simulink library "tip_assist_lib_support"  (Simulink 9.0)
settings: Solver=VariableStepAuto  StartTime=0.0  StopTime=10.0  RelTol=1e-3
undefined symbols (not defined in the file): g, timestep, TipAssistAdvEcmError_t, TipAssistCpmTipOffMode_t, TipAssistLiveWeighStatus_t, TipAssistPayloadType_t, TipAssistSecPfwStatus_t, TipAssistUnsecPfwStatus_t, toa_appNumber, toa_expectedBucketAngNoise, toa_imu_lpf_cutoff_hz, toa_imuBasicOrient, toa_liftBoreDia, toa_liftRodDia, toa_liveLpfCutoffHz, toa_liveSpillRateLpfCutoffHz, toa_mcGroundCombBucketAng, toa_mcGroundCombLiftNormAng, toa_mcGroundLiftNormAng, toa_noSlidingAngle, toa_payload_target_ov_val, toa_payloadTargetMin, toa_pfwLpfCutoffHz, toa_pfwResetLpfCutoffHz, toa_pfwResetStatsBound, toa_pfwResetStatsConf, toa_pfwTiltNormRackThresh, toa_pfwTravelExtentLower, toa_pfwTravelExtentUpper, toa_ratedPayload, toa_reposeMarginAng, toa_sendCpmLiveLpfCutoffHz, toa_sendToCpmMinPrecision, toa_tiltBoreDia, toa_tiltNumCyl, toa_tiltRodDia, toa_toolBcAngle, toa_toolBcLength
libraries: lib_CATutils_Utilities_ApplyName_v2 x113, simulink x18, tip_assist_lib x14, lib_CATutils_Filters_1Pole_LowPass x6, simulink_extras x5, lib_CATutils_Override x3, lib_CATutils_Hysteresis_Latch x3, lib_CATutils_Timer_Countdown x3, tip_assist_lib_support x2
(part 2 of 4)

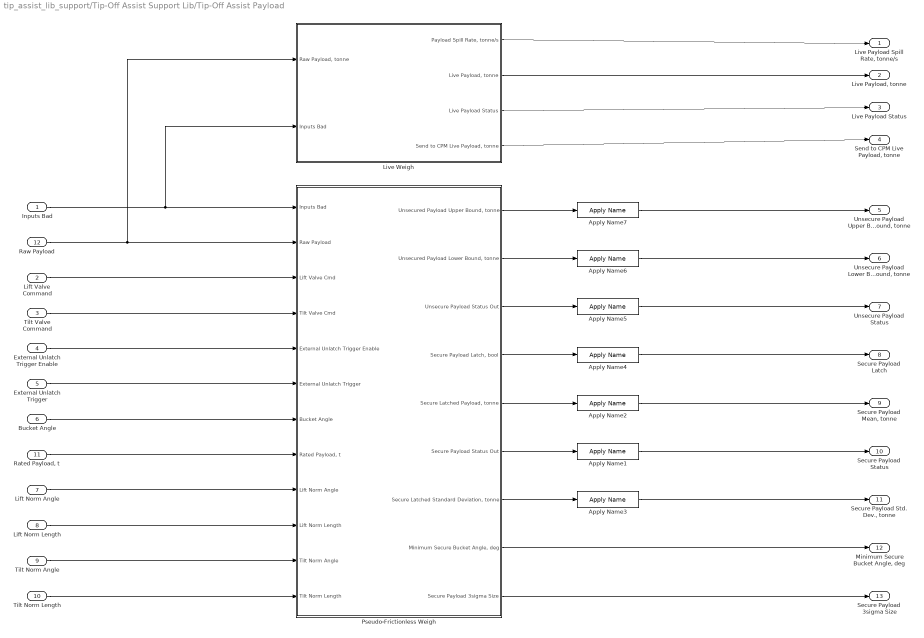
== system tip_assist_lib_support/Tip-Off Assist Support Lib/Tip-Off Assist Payload ==
  Inputs Bad : Inport
  Lift Valve Command : Inport  Port=2
  Tilt Valve Command : Inport  Port=3
  External Unlatch Trigger Enable : Inport  Port=4
  External Unlatch Trigger : Inport  Port=5
  Bucket Angle : Inport  Port=6
  Lift Norm Angle : Inport  Port=7
  Lift Norm Length : Inport  Port=8
  Tilt Norm Angle : Inport  Port=9
  Tilt Norm Length : Inport  Port=10
  "Rated Payload, t" : Inport  Port=11
  Raw Payload : Inport  Port=12
  Apply Name1 : lib_CATutils_Utilities_ApplyName_v2/Apply Name  sigLabel='toa_pfwSecStatus'  enTst=true
  Apply Name2 : lib_CATutils_Utilities_ApplyName_v2/Apply Name  sigLabel='toa_pfwSecPayload'  enTst=true
  Apply Name3 : lib_CATutils_Utilities_ApplyName_v2/Apply Name  sigLabel='toa_pfwSecStDev'  enTst=true
  Apply Name4 : lib_CATutils_Utilities_ApplyName_v2/Apply Name  sigLabel='toa_pfwSecLatch'  enTst=true
  Apply Name5 : lib_CATutils_Utilities_ApplyName_v2/Apply Name  sigLabel='toa_pfwUnsecStatus'  enTst=true
  Apply Name6 : lib_CATutils_Utilities_ApplyName_v2/Apply Name  sigLabel='toa_pfwUnsecBoundLower'  enTst=true
  Apply Name7 : lib_CATutils_Utilities_ApplyName_v2/Apply Name  sigLabel='toa_pfwUnsecBoundUpper'  enTst=true
  Live Weigh : Subsystem
  Pseudo-Frictionless Weigh : Subsystem
  "Live Payload Spill Rate, tonne/s" : Outport
  "Live Payload, tonne" : Outport  Port=2
  Live Payload Status : Outport  Port=3
  "Send to CPM Live Payload, tonne" : Outport  Port=4
  "Unsecure Payload Upper Bound, tonne" : Outport  Port=5
  "Unsecure Payload Lower Bound, tonne" : Outport  Port=6
  Unsecure Payload Status : Outport  Port=7
  Secure Payload Latch : Outport  Port=8
  "Secure Payload Mean, tonne" : Outport  Port=9
  Secure Payload Status : Outport  Port=10
  "Secure Payload Std. Dev., tonne" : Outport  Port=11
  "Minimum Secure Bucket Angle, deg" : Outport  Port=12
  Secure Payload 3sigma Size : Outport  Port=13
  wires:
  Lift Valve Command/1 -> Pseudo-Frictionless Weigh/3(Lift Valve Cmd)
  Tilt Valve Command/1 -> Pseudo-Frictionless Weigh/4(Tilt Valve Cmd)
  Pseudo-Frictionless Weigh/7("Secure Latched Standard Deviation, tonne") -> Apply Name3/1
  Pseudo-Frictionless Weigh/6(Secure Payload Status Out) -> Apply Name1/1
  Pseudo-Frictionless Weigh/4("Secure Payload Latch, bool") -> Apply Name4/1
  Pseudo-Frictionless Weigh/5("Secure Latched Payload, tonne") -> Apply Name2/1
  Raw Payload/1 -> Live Weigh/1("Raw Payload, tonne"), Pseudo-Frictionless Weigh/2(Raw Payload)
  Inputs Bad/1 -> Live Weigh/2(Inputs Bad), Pseudo-Frictionless Weigh/1(Inputs Bad)
  Live Weigh/1("Payload Spill Rate, tonne/s") -> "Live Payload Spill Rate, tonne/s"/1
  Live Weigh/2("Live Payload, tonne") -> "Live Payload, tonne"/1
  Live Weigh/3(Live Payload Status) -> Live Payload Status/1
  External Unlatch Trigger Enable/1 -> Pseudo-Frictionless Weigh/5(External Unlatch Trigger Enable)
  External Unlatch Trigger/1 -> Pseudo-Frictionless Weigh/6(External Unlatch Trigger)
  Bucket Angle/1 -> Pseudo-Frictionless Weigh/7(Bucket Angle)
  Pseudo-Frictionless Weigh/2("Unsecured Payload Lower Bound, tonne") -> Apply Name6/1
  Pseudo-Frictionless Weigh/1("Unsecured Payload Upper Bound, tonne") -> Apply Name7/1
  "Rated Payload, t"/1 -> Pseudo-Frictionless Weigh/8("Rated Payload, t")
  Lift Norm Angle/1 -> Pseudo-Frictionless Weigh/9("Lift Norm Angle ")
  Lift Norm Length/1 -> Pseudo-Frictionless Weigh/10(Lift Norm Length)
  Tilt Norm Angle/1 -> Pseudo-Frictionless Weigh/11(Tilt Norm Angle)
  Tilt Norm Length/1 -> Pseudo-Frictionless Weigh/12(Tilt Norm Length)
  Pseudo-Frictionless Weigh/3(Unsecure Payload Status Out) -> Apply Name5/1
  Apply Name4/1 -> Secure Payload Latch/1
  Apply Name2/1 -> "Secure Payload Mean, tonne"/1
  Apply Name1/1 -> Secure Payload Status/1
  Apply Name3/1 -> "Secure Payload Std. Dev., tonne"/1
  Apply Name5/1 -> Unsecure Payload Status/1
  Apply Name6/1 -> "Unsecure Payload Lower Bound, tonne"/1
  Apply Name7/1 -> "Unsecure Payload Upper Bound, tonne"/1
  Pseudo-Frictionless Weigh/8("Minimum Secure Bucket Angle, deg") -> "Minimum Secure Bucket Angle, deg"/1
  Pseudo-Frictionless Weigh/9(Secure Payload 3sigma Size) -> Secure Payload 3sigma Size/1
  Live Weigh/4("Send to CPM Live Payload, tonne") -> "Send to CPM Live Payload, tonne"/1

== system tip_assist_lib_support/Tip-Off Assist Support Lib/EEF IMU to NEEF gravity vector/imu lpf x1 ==
  in : Inport
  "cutoff freq, Hz" : Inport  Port=2
  Filter Factor Calc : Subsystem
  Single Pole Low Pass Filter : lib_CATutils_Filters_1Pole_LowPass/Single Pole Low Pass Filter  extFactor=on  extReset=off  incIntWordSize=off  mainInternalRes=off  filtFactor=.0001
  Single Pole Low Pass Filter1 : lib_CATutils_Filters_1Pole_LowPass/Single Pole Low Pass Filter  extFactor=on  extReset=off  incIntWordSize=off  mainInternalRes=off  filtFactor=.0001
  out : Outport
  wires:
  in/1 -> Single Pole Low Pass Filter/1
  Single Pole Low Pass Filter1/1 -> out/1
  Single Pole Low Pass Filter/1 -> Single Pole Low Pass Filter1/1
  "cutoff freq, Hz"/1 -> Filter Factor Calc/1(Cutoff (Hz))
  Filter Factor Calc/1(Filter Factor) -> Single Pole Low Pass Filter1/2, Single Pole Low Pass Filter/2

== system tip_assist_lib_support/Tip-Off Assist Support Lib/EEF IMU to NEEF gravity vector/normalize vector ==
  in : Inport
  Divide : Product  Inputs=*/  OutDataTypeStr=Inherit: Same as first input
  Math Function : Math  Operator=square  SaturateOnIntegerOverflow=on
  Math Function1 : Math  Operator=sqrt  SaturateOnIntegerOverflow=on
  Sum of Elements : Sum  Inputs=+
  out : Outport
  wires:
  Divide/1 -> out/1
  in/1 -> Math Function/1, Divide/1
  Math Function1/1 -> Divide/2
  Math Function/1 -> Sum of Elements/1
  Sum of Elements/1 -> Math Function1/1

== system tip_assist_lib_support/Tip-Off Assist Support Lib/Gravity Relevant Components/Magnitude ==
  vector : Inport
  Math Function : Math  Operator=square  SaturateOnIntegerOverflow=on
  Math Function1 : Math  Operator=sqrt  SaturateOnIntegerOverflow=on
  Sum of Elements : Sum  Inputs=+
  magnitude : Outport
  wires:
  vector/1 -> Math Function/1
  Sum of Elements/1 -> Math Function1/1
  Math Function/1 -> Sum of Elements/1
  Math Function1/1 -> magnitude/1

== system tip_assist_lib_support/Tip-Off Assist Support Lib/Send to Implement/Arbitrated Payload Fit in Datalink Representation ==
  In : Inport
  Constant : Constant  Value=200  OutDataTypeStr=single  SampleTime=-1
  Relational Operator : RelationalOperator  Operator=isNaN  OutDataTypeStr=boolean  RndMeth=Simplest
  Saturation : Saturate  UpperLimit=200  LowerLimit=-200
  Switch : Switch  Criteria=u2 ~= 0
  Out : Outport
  wires:
  Relational Operator/1 -> Switch/2
  In/1 -> Relational Operator/1, Switch/3
  Constant/1 -> Switch/1
  Switch/1 -> Saturation/1
  Saturation/1 -> Out/1

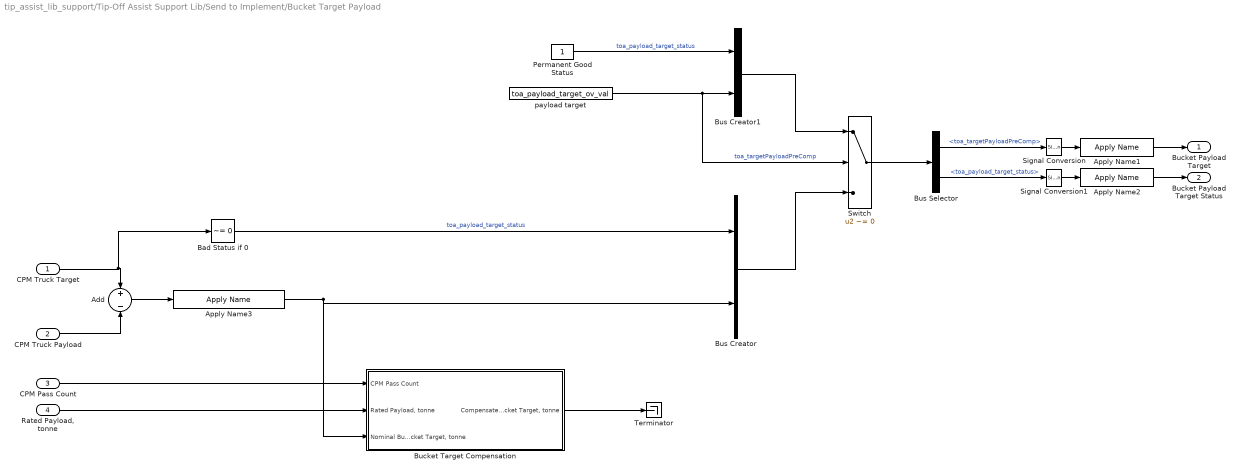
== system tip_assist_lib_support/Tip-Off Assist Support Lib/Send to Implement/Bucket Target Payload ==
  CPM Truck Target : Inport
  CPM Truck Payload : Inport  Port=2
  CPM Pass Count : Inport  Port=3
  "Rated Payload, tonne" : Inport  Port=4
  Add : Sum  Inputs=+-  SaturateOnIntegerOverflow=on  InputSameDT=on  OutDataTypeStr=Inherit: Same as first input
  Apply Name1 : lib_CATutils_Utilities_ApplyName_v2/Apply Name  sigLabel='toa_targetPayloadFinal'  enTst=true
  Apply Name2 : lib_CATutils_Utilities_ApplyName_v2/Apply Name  sigLabel='toa_targetPayloadStatus'  enTst=true
  Apply Name3 : lib_CATutils_Utilities_ApplyName_v2/Apply Name  sigLabel='toa_targetPayloadPreComp'  enTst=true
  Bad Status if 0 : simulink/Logic and Bit Operations/Compare To Constant  relop=~=  const=0  OutDataTypeStr=boolean
      settings: AttributesFormatString=Operator: %<relop>\nConst: %<const>
  Bucket Target Compensation : Subsystem
  Bus Creator : BusCreator  Inputs=2
  Bus Creator1 : BusCreator  Inputs=2
  Bus Selector : BusSelector  OutputSignals=toa_targetPayloadPreComp,toa_payload_target_status
  Permanent Good Status : Constant  OutDataTypeStr=boolean  SampleTime=-1
  Signal Conversion : SignalConversion  OverrideOpt=off
  Signal Conversion1 : SignalConversion  OverrideOpt=off
  Switch : Switch  Criteria=u2 ~= 0  SaturateOnIntegerOverflow=on  InputSameDT=on
      settings: AttributesFormatString=Criteria: %<Criteria>
  Terminator : Terminator
  payload target : Constant  Value=toa_payload_target_ov_val  OutDataTypeStr=single  SampleTime=-1
  Bucket Payload Target : Outport
  Bucket Payload Target Status : Outport  Port=2
  wires:
  Bus Selector/1 -> Signal Conversion/1  "<toa_targetPayloadPreComp>"
  Switch/1 -> Bus Selector/1
  payload target/1 -> Bus Creator1/2, Switch/2  "toa_targetPayloadPreComp"
  Bus Creator1/1 -> Switch/1
  Bus Creator/1 -> Switch/3
  Permanent Good Status/1 -> Bus Creator1/1  "toa_payload_target_status"
  CPM Truck Payload/1 -> Add/2
  Bad Status if 0/1 -> Bus Creator/1  "toa_payload_target_status"
  Add/1 -> Apply Name3/1
  CPM Truck Target/1 -> Add/1, Bad Status if 0/1
  Bus Selector/2 -> Signal Conversion1/1  "<toa_payload_target_status>"
  Signal Conversion/1 -> Apply Name1/1
  Signal Conversion1/1 -> Apply Name2/1
  Apply Name1/1 -> Bucket Payload Target/1
  Apply Name2/1 -> Bucket Payload Target Status/1
  CPM Pass Count/1 -> Bucket Target Compensation/1(CPM Pass Count)
  "Rated Payload, tonne"/1 -> Bucket Target Compensation/2("Rated Payload, tonne")
  Bucket Target Compensation/1("Compensated Bucket Target, tonne") -> Terminator/1
  Apply Name3/1 -> Bucket Target Compensation/3("Nominal Bucket Target, tonne"), Bus Creator/2

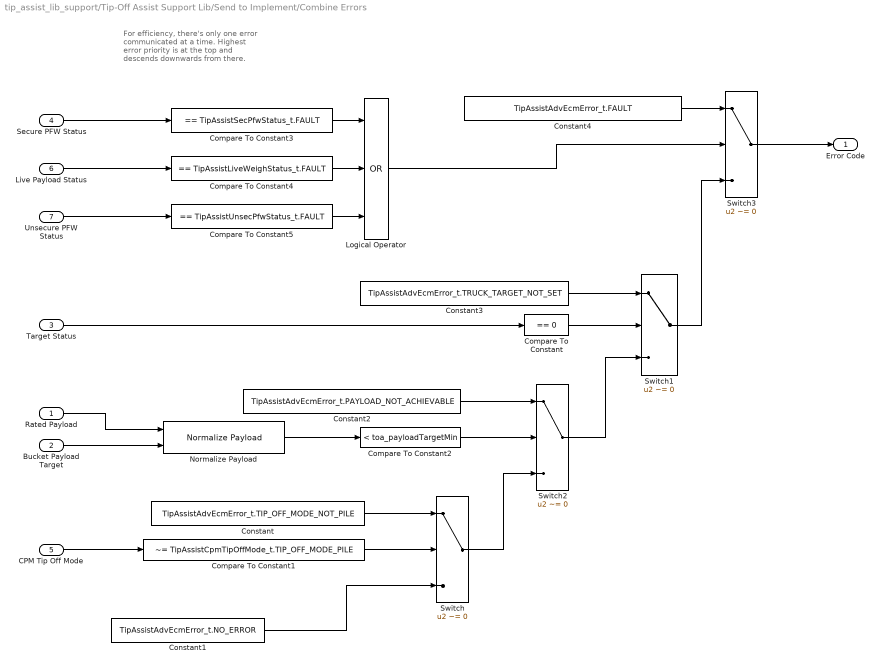
== system tip_assist_lib_support/Tip-Off Assist Support Lib/Send to Implement/Combine Errors ==
  note: For efficiency, there's only one error communicated at a time. Highest error priority is at the top and descends downwards from there.
  Rated Payload : Inport
  Bucket Payload Target : Inport  Port=2
  Target Status : Inport  Port=3
  Secure PFW Status : Inport  Port=4
  CPM Tip Off Mode : Inport  Port=5
  Live Payload Status : Inport  Port=6
  Unsecure PFW Status : Inport  Port=7
  Compare To Constant : simulink/Logic and Bit Operations/Compare To Constant  relop===  const=0  OutDataTypeStr=boolean
  Compare To Constant1 : simulink/Logic and Bit Operations/Compare To Constant  relop=~=  const=TipAssistCpmTipOffMode_t.TIP_OFF_MODE_PILE  OutDataTypeStr=boolean
  Compare To Constant2 : simulink/Logic and Bit Operations/Compare To Constant  relop=<  const=toa_payloadTargetMin  OutDataTypeStr=boolean
  Compare To Constant3 : simulink/Logic and Bit Operations/Compare To Constant  relop===  const=TipAssistSecPfwStatus_t.FAULT  OutDataTypeStr=boolean
  Compare To Constant4 : simulink/Logic and Bit Operations/Compare To Constant  relop===  const=TipAssistLiveWeighStatus_t.FAULT  OutDataTypeStr=boolean
  Compare To Constant5 : simulink/Logic and Bit Operations/Compare To Constant  relop===  const=TipAssistUnsecPfwStatus_t.FAULT  OutDataTypeStr=boolean
  Constant : Constant  Value=TipAssistAdvEcmError_t.TIP_OFF_MODE_NOT_PILE  SampleTime=-1
  Constant1 : Constant  Value=TipAssistAdvEcmError_t.NO_ERROR  SampleTime=-1
  Constant2 : Constant  Value=TipAssistAdvEcmError_t.PAYLOAD_NOT_ACHIEVABLE  SampleTime=-1
  Constant3 : Constant  Value=TipAssistAdvEcmError_t.TRUCK_TARGET_NOT_SET  SampleTime=-1
  Constant4 : Constant  Value=TipAssistAdvEcmError_t.FAULT  SampleTime=-1
  Logical Operator : Logic  Operator=OR  Inputs=3  AllPortsSameDT=off  OutDataTypeStr=boolean
  Normalize Payload : tip_assist_lib/Normalize Payload
  Switch{,1..3} (4 alike) : Switch  Criteria=u2 ~= 0
  Error Code : Outport
  wires:
  Constant/1 -> Switch/1
  CPM Tip Off Mode/1 -> Compare To Constant1/1
  Compare To Constant/1 -> Switch1/2
  Compare To Constant1/1 -> Switch/2
  Target Status/1 -> Compare To Constant/1
  Constant3/1 -> Switch1/1
  Constant1/1 -> Switch/3
  Bucket Payload Target/1 -> Normalize Payload/2
  Constant2/1 -> Switch2/1
  Compare To Constant2/1 -> Switch2/2
  Normalize Payload/1 -> Compare To Constant2/1
  Switch3/1 -> Error Code/1
  Live Payload Status/1 -> Compare To Constant4/1
  Secure PFW Status/1 -> Compare To Constant3/1
  Compare To Constant3/1 -> Logical Operator/1
  Compare To Constant4/1 -> Logical Operator/2
  Logical Operator/1 -> Switch3/2
  Constant4/1 -> Switch3/1
  Rated Payload/1 -> Normalize Payload/1
  Switch1/1 -> Switch3/3
  Switch/1 -> Switch2/3
  Switch2/1 -> Switch1/3
  Unsecure PFW Status/1 -> Compare To Constant5/1
  Compare To Constant5/1 -> Logical Operator/3

== system tip_assist_lib_support/Tip-Off Assist Support Lib/Send to Implement/Payload Multiplexing ==
  Live Payload : Inport
  PFW Latch Status : Inport  Port=2
  PFW Payload : Inport  Port=3
  Constant : Constant  Value=TipAssistPayloadType_t.LIVE  SampleTime=-1
  Constant1 : Constant  Value=TipAssistPayloadType_t.PSEUDO_FRICTIONLESS  SampleTime=-1
  Indexed switch : MultiPortSwitch  DataPortOrder=Zero-based contiguous  Inputs=2  OutDataTypeStr=Inherit: Inherit via back propagation  RndMeth=Nearest  SaturateOnIntegerOverflow=on  InputSameDT=on
  Switch : Switch  Criteria=u2 ~= 0
  Tip-Off Assist Payload Type : Outport
  Tip-Off Assist Payload : Outport  Port=2
  wires:
  PFW Payload/1 -> Switch/1
  PFW Latch Status/1 -> Switch/2, Indexed switch/1
  Live Payload/1 -> Switch/3
  Indexed switch/1 -> Tip-Off Assist Payload Type/1
  Switch/1 -> Tip-Off Assist Payload/1
  Constant1/1 -> Indexed switch/3
  Constant/1 -> Indexed switch/2

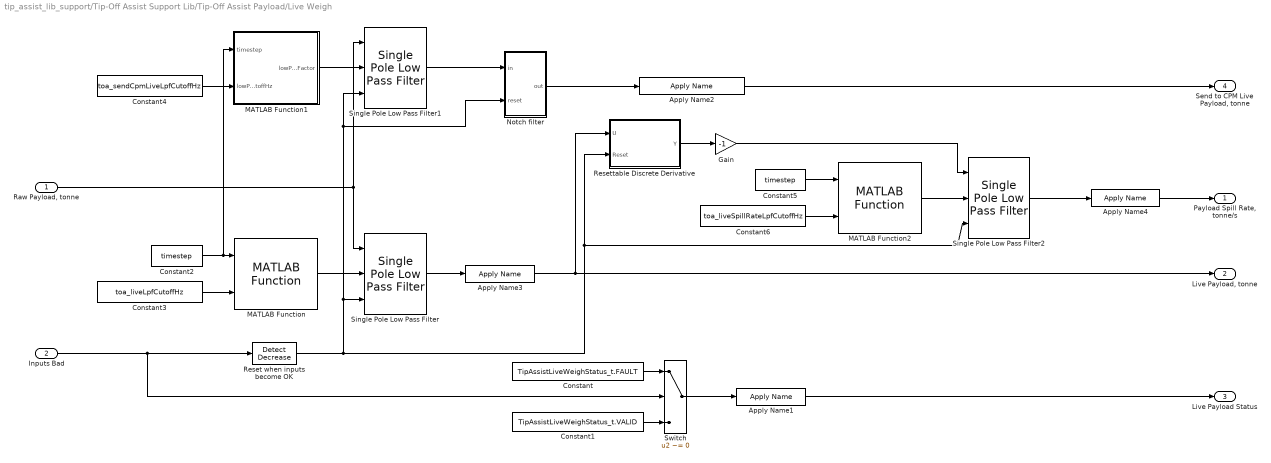
== system tip_assist_lib_support/Tip-Off Assist Support Lib/Tip-Off Assist Payload/Live Weigh ==
  "Raw Payload, tonne" : Inport
  Inputs Bad : Inport  Port=2
  Apply Name1 : lib_CATutils_Utilities_ApplyName_v2/Apply Name  sigLabel='toa_lwStatus'  enTst=true
  Apply Name2 : lib_CATutils_Utilities_ApplyName_v2/Apply Name  sigLabel='toa_sendCpmLivePayload'  enTst=true
  Apply Name3 : lib_CATutils_Utilities_ApplyName_v2/Apply Name  sigLabel='toa_lwLpfPost'  enTst=true
  Apply Name4 : lib_CATutils_Utilities_ApplyName_v2/Apply Name  sigLabel='toa_lwSpillRate'  enTst=true
  Constant : Constant  Value=TipAssistLiveWeighStatus_t.FAULT  SampleTime=-1
  Constant1 : Constant  Value=TipAssistLiveWeighStatus_t.VALID  SampleTime=-1
  Constant2 : Constant  Value=timestep  SampleTime=timestep
  Constant3 : Constant  Value=toa_liveLpfCutoffHz  SampleTime=timestep
  Constant4 : Constant  Value=toa_sendCpmLiveLpfCutoffHz  SampleTime=timestep
  Constant5 : Constant  Value=timestep  SampleTime=timestep
  Constant6 : Constant  Value=toa_liveSpillRateLpfCutoffHz  SampleTime=timestep
  Gain : Gain  Gain=-1
  MATLAB Function : tip_assist_lib/MATLAB Function
      settings: SourceProductName=Stateflow  SourceProductBaseCode=SF
  MATLAB Function1 : MATLAB Function  TreatAsAtomicUnit=on
  MATLAB Function2 : tip_assist_lib/MATLAB Function
      settings: SourceProductName=Stateflow  SourceProductBaseCode=SF
  Notch filter : Subsystem
  Reset when inputs become OK : simulink/Logic and Bit Operations/Detect Decrease  vinit=0  OutDataTypeStr=boolean
  Resettable Discrete Derivative : Subsystem  mask(Discrete Derivative){gainval=1, InputProcessing=Inherited, OutMin=[], OutMax=[], OutDataTypeStr=single, OutputDataTypeScalingMode=single, OutDataType=fixdt(1, 16), OutScaling=2^-10, LockScale=off, RndMeth=Floor, DoSatur=off}
      mask prompts: gainval "Simulink:masks:GainValue_MP"; InputProcessing "Simulink:masks:InputProcessing_MP"; OutMin "Simulink:masks:OutputMinimum_MP"; OutMax "Simulink:masks:OutputMaximum_MP"; OutDataTypeStr "Simulink:masks:OutputDataType_MP"; OutputDataTypeScalingMode "Simulink:masks:OutputDataTypeMode_MP"; OutDataType "Simulink:masks:OutputDataTypeegFixdt116Fixdtsingle_MP"; OutScaling "Simulink:masks:OutputScalingSlopeEg29OrSlopeBias_MP"; LockScale "Simulink:masks:LockOutputDataTypeAgainstFxpTools_MP"; RndMeth "Simulink:masks:IntegerRoundingMode_MP"; DoSatur "Simulink:masks:SaturateToMaxOrMinWhenOverflowsOccur_MP"
      mask help: Simulink:masks:DiscreteDerivative_MD
      mask init:
      | blkH = gcbh;
      | blkName = getfullname(blkH);
      | 
      | if (gainval == 0.0)
      |     %avoid divide by zero warning
      |     inverseGainval = inf;
      | else
      |     inverseGainval = 1.0/double(gainval);
      | end
      | 
      | if isequal(OutDataTypeStr, 'Inherit: Inherit via internal rule')
      |     diffDT   = 'Inherit: Inherit via back propagation';
      |     tsampDT  = 'Inherit: Inherit via internal rule';
      |     tsampImp = 'Offline Scaling Adjustment';
      | else    
      |     diffDT   = OutDataTypeStr;
      |     tsampDT  = 'Inherit: Inherit via back propagation';
      |     tsampImp = 'Online Calculations';
      | end
      | 
      | if ~strcmp(get_param(bdroot(blkH),'SimulationStatus'), 'running')
      |     set_param([blkName,'/Diff'], ...
      |               'RndMeth',RndMeth, ...
      | 	          'DoSatur',DoSatur);
      |     set_param([blkName,'/TSamp'], ...
      |               'OutDataTypeStr',tsampDT, ...
      |               'RndMeth',RndMeth, ...
      |               'DoSatur',DoSatur, ...
      |               'TsampMathImp',tsampImp);
      | end
      | 
      | set_param([blkName,'/Resettable Delay'], ...
      | 	'InputProcessing',InputProcessing);
      mask TypeOptions InputProcessing: Simulink:masks:ColumnsAsChannelsFrameBased | Simulink:masks:ElementsAsChannelsSampleBased | Simulink:masks:Inherited
      mask Callback OutDataTypeStr: fixptdialog(gcbh)
      mask TypeOptions OutputDataTypeScalingMode: double | single | int8 | uint8 | int16 | uint16 | int32 | uint32 | Specify via dialog | Inherit via internal rule | Inherit via back propagation
      mask Callback OutputDataTypeScalingMode: fixptdialog(gcbh)
      mask Callback OutDataType: fixptdialog(gcbh)
      mask TypeOptions RndMeth: Simulink:masks:Ceiling | Simulink:masks:Convergent | Simulink:masks:Floor | Simulink:masks:Nearest | Simulink:masks:Round | Simulink:masks:Simplest | Simulink:masks:Zero
      mask Display: text(0.5, 0.5, 'K (z-1)', 'horizontalAlignment', 'center', 'verticalAlignment', 'bottom');text(0.5, 0.5, 'Ts z', 'horizontalAlignment', 'center', 'verticalAlignment', 'top');plot([0.3 0.7],[0.5 0.5]);
  Single Pole Low Pass Filter : lib_CATutils_Filters_1Pole_LowPass/Single Pole Low Pass Filter  extFactor=on  extReset=on  incIntWordSize=off  mainInternalRes=off  filtFactor=.0001
  Single Pole Low Pass Filter1 : lib_CATutils_Filters_1Pole_LowPass/Single Pole Low Pass Filter  extFactor=on  extReset=on  incIntWordSize=off  mainInternalRes=off  filtFactor=.0001
  Single Pole Low Pass Filter2 : lib_CATutils_Filters_1Pole_LowPass/Single Pole Low Pass Filter  extFactor=on  extReset=on  incIntWordSize=off  mainInternalRes=off  filtFactor=.0001
  Switch : Switch  Criteria=u2 ~= 0
  "Payload Spill Rate, tonne/s" : Outport
  "Live Payload, tonne" : Outport  Port=2
  Live Payload Status : Outport  Port=3
  "Send to CPM Live Payload, tonne" : Outport  Port=4
  wires:
  Single Pole Low Pass Filter/1 -> Apply Name3/1
  MATLAB Function/1 -> Single Pole Low Pass Filter/2
  Reset when inputs become OK/1 -> Notch filter/2(reset), Single Pole Low Pass Filter1/3, Single Pole Low Pass Filter/3, Resettable Discrete Derivative/2(Reset), Single Pole Low Pass Filter2/3
  Inputs Bad/1 -> Switch/2, Reset when inputs become OK/1
  "Raw Payload, tonne"/1 -> Single Pole Low Pass Filter/1, Single Pole Low Pass Filter1/1
  Constant/1 -> Switch/1
  Constant1/1 -> Switch/3
  Switch/1 -> Apply Name1/1
  Constant2/1 -> MATLAB Function1/1(timestep), MATLAB Function/1
  Constant3/1 -> MATLAB Function/2
  Apply Name1/1 -> Live Payload Status/1
  Resettable Discrete Derivative/1(Y) -> Gain/1
  Gain/1 -> Single Pole Low Pass Filter2/1
  Apply Name3/1 -> Resettable Discrete Derivative/1(U), "Live Payload, tonne"/1
  Apply Name4/1 -> "Payload Spill Rate, tonne/s"/1
  MATLAB Function1/1(lowPassFilterFactor) -> Single Pole Low Pass Filter1/2
  Constant4/1 -> MATLAB Function1/2(lowPassFilterCutoffHz)
  Single Pole Low Pass Filter1/1 -> Notch filter/1(in)
  Notch filter/1(out) -> Apply Name2/1
  Apply Name2/1 -> "Send to CPM Live Payload, tonne"/1
  MATLAB Function2/1 -> Single Pole Low Pass Filter2/2
  Constant6/1 -> MATLAB Function2/2
  Constant5/1 -> MATLAB Function2/1
  Single Pole Low Pass Filter2/1 -> Apply Name4/1

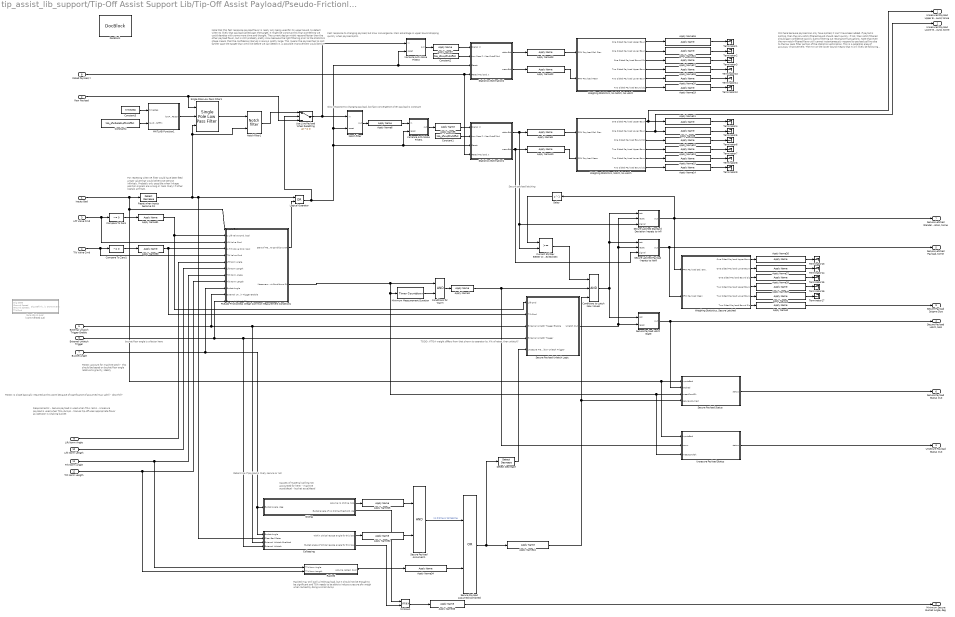
== system tip_assist_lib_support/Tip-Off Assist Support Lib/Tip-Off Assist Payload/Pseudo-Frictionless Weigh ==
  note: Racked may still spill a little payload, but it should not be enough to be significant and TOA needs to be able to induce a secure pfw weigh when racked by doing a small dump
  note: Note that this fast response payload flavor is really only being used for its upper bound, to detect when its likely that payload spilled past the target. It might be worse at this than something we could develop with some more time and thought. The current design might respond faster than the other payload flavor, but is still probably pretty slow because the light filtering prior to the statistics stage means that the confidence interval is always pretty large. This means the payload has to spill farther past the target than we'd like before we can detect it. A possible improvement would be to replace the fast response payload flavor with something faster. One idea is to use the secure payload flavor's upper bound minus some estimate of spilling that is based on live payload. Or, an estimate of spilling that is based on some bespoke algorithm on live payload such as peak and trough detection and processing.
  note: MIN here because payload can only have spilled, it can't have been added.
      |
      | If paylod is spilling, then the non-notch-filtered bound should react quickly.  If not, then notch filtered should gain confidence quickly due to filtering out resonance fluctuations.
      |
      | Note that even the non-notch-filtered flavor still cannot instantaneously respond to payload spilling due to the low pass filter portion of the statistics estimation.  This is a potential area of accuracy improvement.
      |
      | The min on the lower bound means that it will likely be following the non-notch-filtered lower bound because that one converges slower and so will stay lower longer.  This means we will be slower to recognize that payload is above target.  That's acceptable because:
      | 1. TOA will tip again if we don't reach a conclusion about what to do and the measurement period ends
      | 2. The bound is more conservative, reflecting our uncertainty about how much payload might have spilled.  This is important for estimation of the dump increment in the implement control.  If we incorrectly think that our lower bound is higher, we will think we can dump through a larger angle to spill more payload in the next tip increment.
  note: Determine if payload is likely secure or not
  note: Secure payload latching
  note: Fast response to changing payload, but slow convergence. Main advantage is upper bound dropping quickly when payload spills.
  note: Slow response to changing payload, but fast convergence when payload is constant
  note: For resetting when IIR filter could have been feed a NaN value that would otherwise persist infinitely. Probably only possible when linkage position signals are wrong or (less likely) if other signals are NaN.
  note: TODO: account for machine pitch - this should be based on bucket floor angle relative to gravity, ideally
  note: bucket floor angle is a factor here
  note: Causes of material spilling not accounted for here:
      | - machine accel/decel
      | - bucket accel/decel
  note: Requirements:
      | - Secure payload is used when TOA racks
      | - Unsecure payload is used when TOA dumps
      | - Manual tip-off uses appropriate flavor as operator is shaking bucket
  note: TODO: if TOA weight differs from that shown to operator by X% of rated, then unlatch?
  note: TODO: Is slope basically required at this point because of significance of assumed max uphill - downhill?
  Inputs Bad : Inport
  Raw Payload : Inport  Port=2
  Lift Valve Cmd : Inport  Port=3
  Tilt Valve Cmd : Inport  Port=4
  External Unlatch Trigger Enable : Inport  Port=5
  External Unlatch Trigger : Inport  Port=6
  Bucket Angle : Inport  Port=7
  "Rated Payload, t" : Inport  Port=8
  "Lift Norm Angle " : Inport  Port=9
  Lift Norm Length : Inport  Port=10
  Tilt Norm Angle : Inport  Port=11
  Tilt Norm Length : Inport  Port=12
  Apply Name1 : lib_CATutils_Utilities_ApplyName_v2/Apply Name  sigLabel='toa_statPayloadSecureTwoLower'  enTst=true
  Apply Name10 : lib_CATutils_Utilities_ApplyName_v2/Apply Name  sigLabel='toa_pfwNlNotchMeanEst'  enTst=true
  Apply Name11 : lib_CATutils_Utilities_ApplyName_v2/Apply Name  sigLabel='toa_statPayloadNlNotchOneUp'  enTst=true
  Apply Name12 : lib_CATutils_Utilities_ApplyName_v2/Apply Name  sigLabel='toa_statPayloadNlNotchOneSize'  enTst=true
  Apply Name13 : lib_CATutils_Utilities_ApplyName_v2/Apply Name  sigLabel='toa_statPayloadNlNotchTwoUp'  enTst=true
  Apply Name14 : lib_CATutils_Utilities_ApplyName_v2/Apply Name  sigLabel='toa_statPayloadNlNotchTwoSize'  enTst=true
  Apply Name15 : lib_CATutils_Utilities_ApplyName_v2/Apply Name  sigLabel='toa_statPayloadNlNotchTwoLow'  enTst=true
  Apply Name16 : lib_CATutils_Utilities_ApplyName_v2/Apply Name  sigLabel='toa_statPayloadNlOneUp'  enTst=true
  Apply Name17 : lib_CATutils_Utilities_ApplyName_v2/Apply Name  sigLabel='toa_statPayloadNlOneSize'  enTst=true
  Apply Name18 : lib_CATutils_Utilities_ApplyName_v2/Apply Name  sigLabel='toa_statPayloadNlTwoUp'  enTst=true
  Apply Name19 : lib_CATutils_Utilities_ApplyName_v2/Apply Name  sigLabel='toa_statPayloadNlTwoSize'  enTst=true
  Apply Name2 : lib_CATutils_Utilities_ApplyName_v2/Apply Name  sigLabel='toa_statPayloadSecureTwoSize'  enTst=true
  Apply Name20 : lib_CATutils_Utilities_ApplyName_v2/Apply Name  sigLabel='toa_statPayloadNlTwoLow'  enTst=true
  Apply Name21 : lib_CATutils_Utilities_ApplyName_v2/Apply Name  sigLabel='toa_statPayloadNlOneLow'  enTst=true
  Apply Name22 : lib_CATutils_Utilities_ApplyName_v2/Apply Name  sigLabel='toa_pfwNlMeanEst'  enTst=true
  Apply Name23 : lib_CATutils_Utilities_ApplyName_v2/Apply Name  sigLabel='toa_pfwNlStDevEst'  enTst=true
  Apply Name24 : lib_CATutils_Utilities_ApplyName_v2/Apply Name  sigLabel='toa_pfwSecIsSecure'  enTst=true
  Apply Name25 : lib_CATutils_Utilities_ApplyName_v2/Apply Name  sigLabel='toa_pfwSecIsNoSliding'  enTst=true
  Apply Name26 : lib_CATutils_Utilities_ApplyName_v2/Apply Name  sigLabel='toa_statPayloadSecureOneUpper'  enTst=true
  Apply Name27 : lib_CATutils_Utilities_ApplyName_v2/Apply Name  sigLabel='toa_statPayloadSecureOneLower'  enTst=true
  Apply Name28 : lib_CATutils_Utilities_ApplyName_v2/Apply Name  sigLabel='toa_statPayloadSecureOneSize'  enTst=true
  Apply Name29 : lib_CATutils_Utilities_ApplyName_v2/Apply Name  sigLabel='toa_statPayloadSecureTwoUpper'  enTst=true
  Apply Name3 : lib_CATutils_Utilities_ApplyName_v2/Apply Name  sigLabel='toa_pfwIsWarm'  enTst=true
  Apply Name30 : lib_CATutils_Utilities_ApplyName_v2/Apply Name  sigLabel='toa_isTiltValveCmd'  enTst=true
  Apply Name31 : lib_CATutils_Utilities_ApplyName_v2/Apply Name  sigLabel='toa_isLiftValveCmd'  enTst=true
  Apply Name32 : lib_CATutils_Utilities_ApplyName_v2/Apply Name  sigLabel='toa_pfwSecIsNoCollapsing'  enTst=true
  Apply Name33 : lib_CATutils_Utilities_ApplyName_v2/Apply Name  sigLabel='toa_pfwSecMinBucketAng'  enTst=true
  Apply Name34 : lib_CATutils_Utilities_ApplyName_v2/Apply Name  sigLabel='toa_pfwSecIsRacked'  enTst=true
  Apply Name5 : lib_CATutils_Utilities_ApplyName_v2/Apply Name  sigLabel='toa_pfwPayloadNotchFiltFinal'  enTst=true
  Apply Name6 : lib_CATutils_Utilities_ApplyName_v2/Apply Name  sigLabel='toa_pfwPayloadNotchPost'  enTst=true
  Apply Name7 : lib_CATutils_Utilities_ApplyName_v2/Apply Name  sigLabel='toa_pfwPayloadFiltFinal'  enTst=true
  Apply Name8 : lib_CATutils_Utilities_ApplyName_v2/Apply Name  sigLabel='toa_statPayloadNlNotchOneLow'  enTst=true
  Apply Name9 : lib_CATutils_Utilities_ApplyName_v2/Apply Name  sigLabel='toa_pfwNlNotchStDevEst'  enTst=true
  Collapsing : Subsystem
  Compare To Zero : simulink/Logic and Bit Operations/Compare To Zero  relop=~=  OutDataTypeStr=boolean
  Compare To Zero1 : simulink/Logic and Bit Operations/Compare To Zero  relop=~=  OutDataTypeStr=boolean
  Conditions for Warm : Logic
  Conditions to Latch New Values : Logic  Inputs=3
  Constant1 : Constant  Value=toa_pfwLpfCutoffHz
  Constant2 : Constant  Value=toa_pfwLpfCutoffHz
  Constant3 : Constant  Value=timestep  SampleTime=timestep
  Constant4 : Constant  Value=toa_pfwResetLpfCutoffHz  SampleTime=timestep
  Current Std Dev Better or Equal to Previously Latched Std Dev : RelationalOperator  RndMeth=Nearest  InputSameDT=on
  Delay : Delay  DelayLength=1
  Detect Decrease : simulink/Logic and Bit Operations/Detect Decrease  vinit=0.0  OutDataTypeStr=boolean
  DocBlock : simulink/Model-Wide Utilities/DocBlock  DocumentType=Text
      content=|
      | The algorithm stages here:
      | 	• Measurement conditions - is it OK to measure at all?
      |     • Secure vs. unsecure - when to assume each
      | 	• Latch, during measurement
      | 		○ Secure measurement is allowed to continuously latch while measuring
      | 		○ Unsecure does not latch, since material could spill after measurement such as when racking after measurement
      | 	• Latch, post-measurement, "hold on to good data as long as we can"
      | 		○ Most important for Tip-Off Assist
      | 		○ When to replace with more recent, but potentially lower confidence measurements?
      | 			§ If we can unlatch reliably, only replace when confidence is better
      | 			§ If we can't unlatch reliably, always replace
      | 	• Unlatching - when to unlatch
      |         ○ Key principle: When unsure, unlatch!
  Logical Operator : Logic  Operator=OR  AllPortsSameDT=off  OutDataTypeStr=boolean
  MATLAB Function1 : MATLAB Function  TreatAsAtomicUnit=on
  MinMax1 : MinMax  Function=max  Inputs=2
  Minimum Measurement Duration : lib_CATutils_Timer_Countdown/Timer Countdown  initTime=toa_pfw_min_meas_duration  maxTime=400  timingInput=True  expiredOutput=True  initState=False
  Notch filter : Subsystem
  Notch filter1 : tip_assist_lib_support/Tip-Off Assist Support Lib/Tip-Off Assist Payload/Live Weigh/Notch filter
  Pseudo-Frictionless Weigh Common Measurement Conditions : Subsystem
  Racked : Subsystem
  Reset when inputs become OK : simulink/Logic and Bit Operations/Detect Decrease  vinit=0  OutDataTypeStr=boolean
  Secure Latched Payload (resets to NaN) : Subsystem  mask{mskInitialOut=NaN}
      mask prompts: mskInitialOut "Initial Output and Reset Value"
  Secure Latched Standard Deviation (resets to inf) : Subsystem  mask{mskInitialOut=single(inf)}
      mask prompts: mskInitialOut "Initial Output and Reset Value"
  Secure Payload Assumed 1 : Logic  AllPortsSameDT=off  OutDataTypeStr=boolean
  Secure Payload Assumed Combined : Logic  Operator=OR  AllPortsSameDT=off  OutDataTypeStr=boolean
  Secure Payload Latch State : Subsystem  mask{mskInitialOut=0}
      mask prompts: mskInitialOut "Initial Output"
  Secure Payload Status : MATLAB Function  TreatAsAtomicUnit=on
  Secure Payload Unlatch Logic : Subsystem
  Single Pole Low Pass Filter1 : lib_CATutils_Filters_1Pole_LowPass/Single Pole Low Pass Filter  extFactor=on  extReset=on  incIntWordSize=off  mainInternalRes=off  filtFactor=.0001
  Sliding : Subsystem
  Statistics Estimation1 : Subsystem
  Statistics Estimation2 : Subsystem
  Sure dig is over : Subsystem  Commented=on
  Terminator{1..17} (17 alike) : Terminator
  Unsecure Payload Status : MATLAB Function  TreatAsAtomicUnit=on
  Use Live Payload When Resetting : Switch  Criteria=u2 ~= 0
  Variance Anti-Noise Filter1 : Subsystem
  Variance Anti-Noise Filter2 : Subsystem
  "Weighing Statistics, No Notch, No Latch" : Subsystem
  "Weighing Statistics, Notch, No Latch" : Subsystem
  "Weighing Statistics, Secure Latched" : Subsystem
  "Unsecured Payload Upper Bound, tonne" : Outport
  "Unsecured Payload Lower Bound, tonne" : Outport  Port=2
  Unsecure Payload Status Out : Outport  Port=3
  "Secure Payload Latch, bool" : Outport  Port=4
  "Secure Latched Payload, tonne" : Outport  Port=5
  Secure Payload Status Out : Outport  Port=6
  "Secure Latched Standard Deviation, tonne" : Outport  Port=7
  "Minimum Secure Bucket Angle, deg" : Outport  Port=8
  Secure Payload 3sigma Size : Outport  Port=9
  wires:
  Pseudo-Frictionless Weigh Common Measurement Conditions/2(Measurement Conditions OK) -> Conditions for Warm/1, Unsecure Payload Status/3(measCondOk), Secure Payload Status/3(measCondOk), Minimum Measurement Duration/1
  Statistics Estimation1/1(stdevEst) -> Apply Name9/1, Current Std Dev Better or Equal to Previously Latched Std Dev/2, Secure Latched Standard Deviation (resets to inf)/3(signal)
  Secure Payload Status/1(status) -> Secure Payload Status Out/1
  Secure Latched Standard Deviation (resets to inf)/1(out) -> Delay/1, "Weighing Statistics, Secure Latched"/1(PFW Payload Std. Dev.), "Secure Latched Standard Deviation, tonne"/1
  Secure Latched Payload (resets to NaN)/1(out) -> "Weighing Statistics, Secure Latched"/2(PFW Payload Mean), "Secure Latched Payload, tonne"/1
  Apply Name30/1 -> Pseudo-Frictionless Weigh Common Measurement Conditions/4("Is Tilt Valve Cmd, bool"), Secure Payload Unlatch Logic/2(Tilt Cmd)
  Pseudo-Frictionless Weigh Common Measurement Conditions/1(Start of Measurement Conditions OK) -> Logical Operator/2
  Delay/1 -> Current Std Dev Better or Equal to Previously Latched Std Dev/1
  Current Std Dev Better or Equal to Previously Latched Std Dev/1 -> Conditions to Latch New Values/1
  Minimum Measurement Duration/1 -> Conditions for Warm/2
  Secure Payload Latch State/1(out) -> "Secure Payload Latch, bool"/1, Secure Payload Status/2(latched)
  Conditions to Latch New Values/1 -> Secure Latched Payload (resets to NaN)/1(set), Secure Latched Standard Deviation (resets to inf)/1(set), Secure Payload Latch State/1(set)
  Apply Name31/1 -> Secure Payload Unlatch Logic/1(Lift Cmd), Pseudo-Frictionless Weigh Common Measurement Conditions/2("Is Lift Valve Cmd, bool")
  Inputs Bad/1 -> Reset when inputs become OK/1, Unsecure Payload Status/1(inputsBad), Secure Payload Status/1(inputsBad), Pseudo-Frictionless Weigh Common Measurement Conditions/1(Inputs Bad)
  Reset when inputs become OK/1 -> Logical Operator/1, Collapsing/2(Clear Bad State), Notch filter1/2, Single Pole Low Pass Filter1/3
  External Unlatch Trigger/1 -> Pseudo-Frictionless Weigh Common Measurement Conditions/12(External Unlatch Trigger), Collapsing/4(External Unlatch), Secure Payload Unlatch Logic/4(External Unlatch Trigger)
  External Unlatch Trigger Enable/1 -> Pseudo-Frictionless Weigh Common Measurement Conditions/11(External Unlatch Trigger Enable), Collapsing/3(External Unlatch Enabled), Secure Payload Unlatch Logic/3(External Unlatch Trigger Enable)
  Statistics Estimation1/2(meanEst) -> Apply Name10/1, Secure Latched Payload (resets to NaN)/3(signal)
  Conditions for Warm/1 -> Apply Name3/1
  Apply Name3/1 -> Unsecure Payload Status/2(warm), Conditions to Latch New Values/2
  Apply Name5/1 -> Statistics Estimation1/1(Signal In)
  "Weighing Statistics, Notch, No Latch"/3(One Sided Payload Bound Size) -> Apply Name12/1
  "Weighing Statistics, Notch, No Latch"/4(Two Sided Payload Upper Bound) -> Apply Name13/1
  "Rated Payload, t"/1 -> Statistics Estimation1/4("Rated Payload, t"), Statistics Estimation2/4("Rated Payload, t")
  "Weighing Statistics, Notch, No Latch"/5(Two Sided Payload Lower Bound) -> Apply Name15/1
  Variance Anti-Noise Filter1/1(out) -> Apply Name5/1
  "Weighing Statistics, Notch, No Latch"/6(Two Sided Payload Bound Size) -> Apply Name14/1
  Apply Name6/1 -> Variance Anti-Noise Filter1/1(in)
  Notch filter/1(out) -> Apply Name6/1
  Constant1/1 -> Statistics Estimation1/2(Low Pass Filter Cutoff (Hz))
  Constant2/1 -> Statistics Estimation2/2(Low Pass Filter Cutoff (Hz))
  Variance Anti-Noise Filter2/1(out) -> Apply Name7/1
  Apply Name7/1 -> Statistics Estimation2/1(Signal In)
  Apply Name9/1 -> "Weighing Statistics, Notch, No Latch"/1(PFW Payload Std. Dev.)
  Apply Name10/1 -> "Weighing Statistics, Notch, No Latch"/2(PFW Payload Mean)
  Apply Name8/1 -> Terminator5/1
  Apply Name11/1 -> Terminator4/1
  Apply Name12/1 -> Terminator6/1
  Apply Name15/1 -> Terminator8/1
  Apply Name13/1 -> Terminator7/1
  Apply Name14/1 -> Terminator9/1
  Apply Name19/1 -> Terminator12/1
  Apply Name18/1 -> Terminator10/1
  Apply Name20/1 -> Terminator11/1
  Apply Name17/1 -> Terminator3/1
  Apply Name16/1 -> Terminator1/1
  Apply Name21/1 -> Terminator2/1
  "Weighing Statistics, No Notch, No Latch"/1(One Sided Payload Upper Bound) -> Apply Name16/1
  "Weighing Statistics, No Notch, No Latch"/6(Two Sided Payload Bound Size) -> Apply Name19/1
  "Weighing Statistics, No Notch, No Latch"/5(Two Sided Payload Lower Bound) -> Apply Name20/1
  "Weighing Statistics, No Notch, No Latch"/4(Two Sided Payload Upper Bound) -> Apply Name18/1
  "Weighing Statistics, No Notch, No Latch"/2(One Sided Payload Lower Bound) -> Apply Name21/1
  "Weighing Statistics, No Notch, No Latch"/3(One Sided Payload Bound Size) -> Apply Name17/1
  Statistics Estimation2/1(stdevEst) -> Apply Name23/1
  Statistics Estimation2/2(meanEst) -> Apply Name22/1
  Apply Name23/1 -> "Weighing Statistics, No Notch, No Latch"/1(PFW Payload Std. Dev.)
  Apply Name22/1 -> "Weighing Statistics, No Notch, No Latch"/2(PFW Payload Mean)
  "Weighing Statistics, Notch, No Latch"/1(One Sided Payload Upper Bound) -> "Unsecured Payload Upper Bound, tonne"/1, Apply Name11/1
  "Weighing Statistics, Notch, No Latch"/2(One Sided Payload Lower Bound) -> "Unsecured Payload Lower Bound, tonne"/1, Apply Name8/1
  Sliding/1("Assume no sliding, bool") -> Apply Name25/1
  Secure Payload Assumed 1/1 -> Secure Payload Assumed Combined/1  "no sliding or collapsing"
  Racked/1("Assume racked, bool") -> Apply Name34/1
  Secure Payload Assumed Combined/1 -> Detect Decrease/1, Apply Name24/1
  Bucket Angle/1 -> Collapsing/1(Bucket Angle), Sliding/1("Bucket Angle, deg"), Pseudo-Frictionless Weigh Common Measurement Conditions/10(Bucket Angle)
  Collapsing/1(Within critical repose angle for this load) -> Apply Name32/1
  Unsecure Payload Status/1(status) -> Unsecure Payload Status Out/1
  Detect Decrease/1 -> Secure Payload Unlatch Logic/5(Unsecure Transition Unlatch Trigger)
  "Lift Norm Angle "/1 -> Pseudo-Frictionless Weigh Common Measurement Conditions/6("Lift Norm Angle ")
  Lift Norm Length/1 -> Pseudo-Frictionless Weigh Common Measurement Conditions/7(Lift Norm Length)
  Tilt Norm Angle/1 -> Racked/1(Tilt Norm Angle), Pseudo-Frictionless Weigh Common Measurement Conditions/8(Tilt Norm Angle)
  Tilt Norm Length/1 -> Racked/2(Tilt Norm Length), Pseudo-Frictionless Weigh Common Measurement Conditions/9(Tilt Norm Length)
  "Weighing Statistics, Secure Latched"/5(Two Sided Payload Lower Bound) -> Apply Name1/1
  "Weighing Statistics, Secure Latched"/2(One Sided Payload Lower Bound) -> Apply Name27/1
  Apply Name29/1 -> Terminator16/1
  "Weighing Statistics, Secure Latched"/4(Two Sided Payload Upper Bound) -> Apply Name29/1
  "Weighing Statistics, Secure Latched"/6(Two Sided Payload Bound Size) -> Apply Name2/1
  "Weighing Statistics, Secure Latched"/3(One Sided Payload Bound Size) -> Apply Name28/1
  Apply Name27/1 -> Terminator14/1
  Apply Name2/1 -> Secure Payload 3sigma Size/1
  Apply Name26/1 -> Terminator13/1
  Apply Name1/1 -> Terminator17/1
  "Weighing Statistics, Secure Latched"/1(One Sided Payload Upper Bound) -> Apply Name26/1
  Apply Name28/1 -> Terminator15/1
  Sliding/2("Bucket angle of no sliding threshold, deg") -> MinMax1/1
  Collapsing/2(Bucket angle of critical repose angle for this load) -> MinMax1/2
  MinMax1/1 -> Apply Name33/1
  Compare To Zero/1 -> Apply Name31/1
  Compare To Zero1/1 -> Apply Name30/1
  Lift Valve Cmd/1 -> Compare To Zero/1, Pseudo-Frictionless Weigh Common Measurement Conditions/3(Lift Valve Cmd)
  Tilt Valve Cmd/1 -> Pseudo-Frictionless Weigh Common Measurement Conditions/5(Tilt Valve Cmd), Compare To Zero1/1
  Apply Name24/1 -> Secure Payload Status/4(secureAssumed), Conditions to Latch New Values/3
  Apply Name25/1 -> Secure Payload Assumed 1/1
  Apply Name32/1 -> Secure Payload Assumed 1/2
  Apply Name33/1 -> "Minimum Secure Bucket Angle, deg"/1
  Apply Name34/1 -> Secure Payload Assumed Combined/2
  Secure Payload Unlatch Logic/1(Unlatch Out) -> Secure Latched Standard Deviation (resets to inf)/2(reset), Secure Latched Payload (resets to NaN)/2(reset), Secure Payload Latch State/2(reset)
  MATLAB Function1/1(lowPassFilterFactor) -> Single Pole Low Pass Filter1/2
  Single Pole Low Pass Filter1/1 -> Notch filter1/1
  Logical Operator/1 -> Statistics Estimation1/3(Reset), Variance Anti-Noise Filter1/2(reset), Notch filter/2(reset), Variance Anti-Noise Filter2/2(reset), Statistics Estimation2/3(Reset), Use Live Payload When Resetting/2
  Constant3/1 -> MATLAB Function1/1(timestep)
  Constant4/1 -> MATLAB Function1/2(lowPassFilterCutoffHz)
  Raw Payload/1 -> Single Pole Low Pass Filter1/1, Use Live Payload When Resetting/3
  Notch filter1/1 -> Use Live Payload When Resetting/1
  Use Live Payload When Resetting/1 -> Variance Anti-Noise Filter2/1(in), Notch filter/1(in)

== system tip_assist_lib_support/Tip-Off Assist Support Lib/EEF IMU to NEEF gravity vector/imu lpf x1/Filter Factor Calc ==
  Cutoff (Hz) : Inport
  Constant1 : Constant  Value=-2 * pi * timestep  OutDataTypeStr=single
  Constant3 : Constant  OutDataTypeStr=single
  Math Function : Math  OutputSignalType=real  SaturateOnIntegerOverflow=on
  Multiply : Product  SaturateOnIntegerOverflow=on  RndMeth=Zero  InputSameDT=on  OutDataTypeStr=Inherit: Same as first input
  Subtract : Sum  Inputs=|+-  SaturateOnIntegerOverflow=on  InputSameDT=on  OutDataTypeStr=Inherit: Same as first input
  Filter Factor : Outport
  wires:
  Cutoff (Hz)/1 -> Multiply/1
  Subtract/1 -> Filter Factor/1
  Constant3/1 -> Subtract/1
  Multiply/1 -> Math Function/1
  Math Function/1 -> Subtract/2
  Constant1/1 -> Multiply/2

== system tip_assist_lib_support/Tip-Off Assist Support Lib/Send to Implement/Bucket Target Payload/Bucket Target Compensation ==
  note: combined precision (1 sigma)
  CPM Pass Count : Inport
  "Rated Payload, tonne" : Inport  Port=2
  "Nominal Bucket Target, tonne" : Inport  Port=3
  Add : Sum
  Apply Name1 : lib_CATutils_Utilities_ApplyName_v2/Apply Name  sigLabel='toa_targetPayloadPostComp'  enTst=true
  Apply Name3 : lib_CATutils_Utilities_ApplyName_v2/Apply Name  sigLabel='toa_targetCompMargin'  enTst=true
  "Exprected CPM Precision (1 sigma), pct of rated payload" : Constant  Value=.01
  "Exprected TOA Measurement Precision (1 sigma), pct of rated payload" : Constant  Value=.02
  Math Function : Math  Operator=square  SaturateOnIntegerOverflow=on
  Math Function1 : Math  Operator=square  SaturateOnIntegerOverflow=on
  Product{,1..3} (4 alike) : Product
  Square Root : Sqrt  SaturateOnIntegerOverflow=on
  Subtract : Sum  Inputs=+-
  TOA Pass Count : Constant
  "Compensated Bucket Target, tonne" : Outport
  wires:
  Square Root/1 -> Apply Name3/1
  Product2/1 -> Math Function1/1
  Product1/1 -> Add/2
  Math Function1/1 -> Product3/2
  "Rated Payload, tonne"/1 -> Product2/2, Product/1
  "Nominal Bucket Target, tonne"/1 -> Subtract/1  "Norminal bucket target"
  "Exprected TOA Measurement Precision (1 sigma), pct of rated payload"/1 -> Product2/1
  Product/1 -> Math Function/1  "precision (1 sigma), tonne"
  Add/1 -> Square Root/1
  TOA Pass Count/1 -> Product3/1
  Product3/1 -> Add/1
  "Exprected CPM Precision (1 sigma), pct of rated payload"/1 -> Product/2
  Math Function/1 -> Product1/1  "variance"
  Subtract/1 -> Apply Name1/1
  CPM Pass Count/1 -> Product1/2
  Apply Name3/1 -> Subtract/2
  Apply Name1/1 -> "Compensated Bucket Target, tonne"/1

== system tip_assist_lib_support/Tip-Off Assist Support Lib/Tip-Off Assist Payload/Live Weigh/Notch filter ==
  in : Inport
  reset : Inport  Port=2
  NotchFilter : Subsystem  mask{mskCutoffFreqRadPerSec=5.0}
      mask prompts: mskCutoffFreqRadPerSec "Cutoff Frequency (rad/s)"
      settings: AttributesFormatString=cf: %<mskCutoffFreqRadPerSec>
  NotchFilter1 : Subsystem  mask{mskCutoffFreqRadPerSec=7.5}
      mask prompts: mskCutoffFreqRadPerSec "Cutoff Frequency (rad/s)"
      settings: AttributesFormatString=cf: %<mskCutoffFreqRadPerSec>
  NotchFilter2 : Subsystem  mask{mskCutoffFreqRadPerSec=12.0}
      mask prompts: mskCutoffFreqRadPerSec "Cutoff Frequency (rad/s)"
      settings: AttributesFormatString=cf: %<mskCutoffFreqRadPerSec>
  out : Outport
  wires:
  NotchFilter/1(filtered) -> NotchFilter1/1(raw)
  NotchFilter1/1(filtered) -> NotchFilter2/1(raw)
  reset/1 -> NotchFilter2/2(reset), NotchFilter1/2(reset), NotchFilter/2(reset)
  in/1 -> NotchFilter/1(raw)
  NotchFilter2/1(filtered) -> out/1

== system tip_assist_lib_support/Tip-Off Assist Support Lib/Tip-Off Assist Payload/Live Weigh/Resettable Discrete Derivative ==
  note: U(k)
  note: ( U(k) - U(k-1) )
  U : Inport
  Reset : Inport  Port=2
  Data Type Duplicate : DataTypeDuplicate  DisableCoverage=on  NumInputPorts=3
  Diff : Sum  Description=Add in CPU  Inputs=+-  OutMin=OutMin  OutMax=OutMax  OutDataTypeStr=diffDT
  Resettable Delay : Delay  DelayLength=1  InitialConditionSource=Input port  ExternalReset=Level hold  InputProcessing=Inherited
      settings: InputPortMap=u0,r5,p4
  TSamp : SampleTimeMath  DisableCoverage=on  TsampMathOp=/  weightValue=inverseGainval  OutDataTypeStr=Inherit: Inherit via back propagation
  Y : Outport  OutMin=OutMin  OutMax=OutMax  InitialOutput=0
  wires:
  TSamp/1 -> Resettable Delay/1, Resettable Delay/3, Data Type Duplicate/2, Diff/1
  Diff/1 -> Data Type Duplicate/1, Y/1
  Resettable Delay/1 -> Data Type Duplicate/3, Diff/2  "U(k-1)"
  U/1 -> TSamp/1
  Reset/1 -> Resettable Delay/2

== system tip_assist_lib_support/Tip-Off Assist Support Lib/Tip-Off Assist Payload/Pseudo-Frictionless Weigh/Collapsing ==
  note: This minimum angle represents the minimum bucket angle that we know does not exceed the payload's critical angle of repose, because the payload has already been to this angle and any material past the critical angle of repose would have already fallen out. This is useful because that same load can be considered secure as long as the current bucket angle is some margin above this angle.
  Bucket Angle : Inport
  Clear Bad State : Inport  Port=2
  External Unlatch Enabled : Inport  Port=3
  External Unlatch : Inport  Port=4
  Add : Sum
  Add2 : Sum
  Current Bucket Angle Lower Than Or Equal To Previous Min Angle : RelationalOperator  Operator=>  RndMeth=Nearest  InputSameDT=on
  Data Type Conversion : DataTypeConversion  OutDataTypeStr=boolean
  Delay2 : Delay  DelayLength=1
  External Unlatch Enabled and Triggered : Logic  AllPortsSameDT=off  OutDataTypeStr=boolean
  Latched Point Hysteresis : lib_CATutils_Hysteresis_Latch/Latched Point Hysteresis  extBreakPoints=on  Min_Break_Point=-0.5  Max_Break_Point=0.5  extValues=off  Lo_Value=0  Hi_Value=1  Out_Mode=unused and invalid  Out_DataType=[]  Out_Scaling=[]  OutDataTypeStr=int8
  Logical Operator : Logic  Operator=OR  AllPortsSameDT=off  OutDataTypeStr=boolean
  Minimum Angle For Current Load (resets to 99) : Subsystem  mask{mskInitialOut=single(99)}
      mask prompts: mskInitialOut "Initial Output and Reset Value"
  New min angle and external unlatch enabled : Logic  AllPortsSameDT=off  OutDataTypeStr=boolean
  "Secure Load Buffer Angle, degrees" : Constant  Value=toa_reposeMarginAng  OutDataTypeStr=single  SampleTime=-1
  "expected bucket angle noise amplitude, deg" : Constant  Value=toa_expectedBucketAngNoise  OutDataTypeStr=single  SampleTime=-1
  Within critical repose angle for this load : Outport
  Bucket angle of critical repose angle for this load : Outport  Port=2
  wires:
  Minimum Angle For Current Load (resets to 99)/1(out) -> Add/1, Delay2/1
  External Unlatch Enabled and Triggered/1 -> Logical Operator/1
  Data Type Conversion/1 -> Within critical repose angle for this load/1
  "expected bucket angle noise amplitude, deg"/1 -> Add2/2
  Add2/1 -> Latched Point Hysteresis/3
  Bucket Angle/1 -> Latched Point Hysteresis/1, Minimum Angle For Current Load (resets to 99)/3(signal), Current Bucket Angle Lower Than Or Equal To Previous Min Angle/2
  Add/1 -> Bucket angle of critical repose angle for this load/1, Add2/1, Latched Point Hysteresis/2
  Latched Point Hysteresis/1 -> Data Type Conversion/1
  Current Bucket Angle Lower Than Or Equal To Previous Min Angle/1 -> New min angle and external unlatch enabled/1
  Logical Operator/1 -> Minimum Angle For Current Load (resets to 99)/2(reset)
  New min angle and external unlatch enabled/1 -> Minimum Angle For Current Load (resets to 99)/1(set)
  Delay2/1 -> Current Bucket Angle Lower Than Or Equal To Previous Min Angle/1
  External Unlatch/1 -> External Unlatch Enabled and Triggered/2
  Clear Bad State/1 -> Logical Operator/2
  External Unlatch Enabled/1 -> External Unlatch Enabled and Triggered/1, New min angle and external unlatch enabled/2
  "Secure Load Buffer Angle, degrees"/1 -> Add/2
